simulink model "Autonomous_Driving_Car_Example1"  (R2022a)
settings: Solver=ode2  StartTime=0.0  StopTime=inf  FixedStep=1/600  RelTol=1e-3  EnableMultiTasking=on
model workspace (MAT data in the model file):
  camera_rate = Simulink.Parameter
  camera_rate.Value = Simulink.data.Expression
  camera_rate.Value.ExpressionString = "qc_get_step_size * ceil(1/60 / qc_get_step_size)"
  camera_rate.DataType = 'auto'
  camera_rate.Complexity = 'real'
  camera_rate.Dimensions = -1
  depth_rate = Simulink.Parameter
  depth_rate.Value = Simulink.data.Expression
  depth_rate.Value.ExpressionString = "qc_get_step_size * ceil(1/100 / qc_get_step_size)"
  depth_rate.DataType = 'auto'
  depth_rate.Complexity = 'real'
  depth_rate.Dimensions = -1
undefined symbols (not defined in the file): gcbh, height, HIL, JPEG, left, qc_get_step_size, top, Video3D, video_display_show, width
libraries: quarc_library x45, simulink x12
(part 1 of 2)
settings Model: SimulationMode=external  ExtModeTrigDuration=10000  Creator=User  LastModifiedBy=Admin
settings SolverCC: AlgebraicLoopSolver=TrustRegion  PositivePriorityOrder=on  AutoInsertRateTranBlk=on
settings DataIOCC: ReturnWorkspaceOutputs=off
settings DebuggingCC: ParameterPrecisionLossMsg=none  UnconnectedInputMsg=warning  UnconnectedOutputMsg=warning  UnconnectedLineMsg=warning  SFMachineParentedDataDiag=warning  ArithmeticOperatorsInVariantConditions=warning
settings HardwareCC: ProdBitPerLong=64  ProdLargestAtomicInteger=LongLong  ProdLargestAtomicFloat=Double  ProdLongLongMode=on  ProdHWDeviceType=ARM Compatible->ARM 64-bit (LP64)
settings SFSimCC: SimUseLocalCustomCode=off  CustomCodeUndefinedFunction=UseInterfaceOnly
settings RTWCC: Description=QUARC Linux Nvidia Target (QCar) Using Toolchain  SystemTargetFile=quarc_linux_nvidia.tlc  TemplateMakefile=quarc_default_tmf  RTWUseLocalCustomCode=off  Toolchain=QUARC linux_nvidia | gmake (64-bit Windows)  BuildConfiguration=Faster Runs
settings STFCustomTargetCC: TargetLangStandard=C99 (ISO)  ConcurrentExecutionCompliant=on  UseToolchainInfoCompliant=on  SystemTargetFile=quarc_linux_nvidia.tlc
settings GRTTargetCC: ParMdlRefBuildCompliant=off  CompOptLevelCompliant=off  CombineOutputUpdateFcns=off  MatFileLogging=off  CPPClassGenCompliant=off  GRTInterface=on  ExtMode=on  ExtModeMexFile=quarc_comm  ExtModeMexArgs='-w -d /tmp -uri %u','tcpip://192.168.2.11:17001'

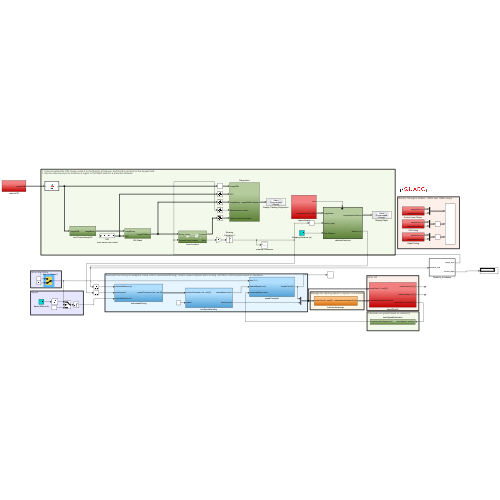
[thumbnail: Simulink's stored preview of the top-level diagram]
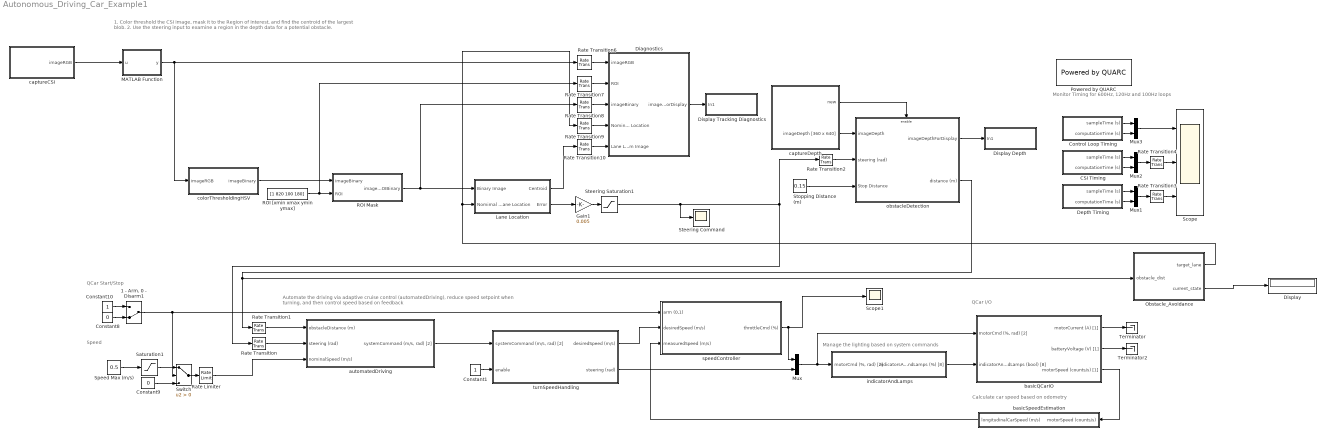
== system Autonomous_Driving_Car_Example1 ==
  note: Monitor Timing for 600Hz, 120Hz and 100Hz loops
  note: Manage the lighting based on system commands
  note: Calculate car speed based on odometry
  note: QCar I/O
  note: Automate the driving via adaptive cruise control (automatedDriving), reduce speed setpoint when turning, and then control speed based on feedback
  note: 1. Color threshold the CSI image, mask it to the Region of Interest, and find the centroid of the largest blob.
      | 2. Use the steering input to examine a region in the depth data for a potential obstacle.
  note: Speed
  note: QCar Start/Stop
  " CSI Timing" : Subsystem
  " Depth Timing" : Subsystem
  "1 - Arm, 0 - Disarm1" : ManualSwitch  CurrentSetting=0
  Constant1 : Constant
  Constant10 : Constant
  Constant8 : Constant  Value=0
  Constant9 : Constant  Value=0
  "Control Loop Timing " : Subsystem
  Diagnostics : Subsystem
  Display : Display
  Display Depth : Subsystem  LoadFcn=set_param(gcbh, 'UserData', gcb);  StartFcn=video_display_show([gcb, '/Video Display'], 'add', gcb);  mask(Video Compressed Display){algorithm=JPEG, quality=50, sample_time=-1, use_hardware=on}
      mask prompts: algorithm "Compression algorithm:"; quality "Compression quality (0-100):"; sample_time "Sample time (seconds):"; use_hardware "Use hardware acceleration for video display"
      mask help: Displays a video stream on the host, using compression to minimize bandwidth.
      mask init:
      | qc_set_display('Video\nCompressed\nDisplay');
      settings: UndoDeleteFcn=set_param(gcbh, 'UserData', gcb);  OpenFcn=video_display_show([gcb, '/Video Display'], 'show', gcb);  PreDeleteFcn=video_display_show([gcb, '/Video Display'], 'delete');
      settings: CopyFcn=|
      | set_param(gcbh, 'UserData', gcb);
      | set_param(gcbh, 'LinkStatus', 'none');
      settings: NameChangeFcn=|
      | video_display_show([get_param(gcbh, 'UserData'), '/Video Display'], 'rename', [gcb, '/Video Display']);
      | video_display_show([gcb, '/Video Display'], 'add', gcb);
      | set_param(gcbh, 'UserData', gcb);
      mask Help: web(qc_get_block_help_path(gcb));
      mask TypeOptions algorithm: Image Compress/algorithm
      mask TypeOptions quality: Image Compress/quality
      mask TypeOptions sample_time: Video Display/sample_time
      mask TypeOptions use_hardware: Video Display/use_hardware
      mask Display:
      | patch([0.98591 0.98591 0.62618 0.59072 0.56147   0.536   0.536  0.5441 0.56912 0.59207 0.60881 0.62276 0.63527 0.64364  0.6485  0.6485 0.64706 0.64499 0.63662 0.62411 0.61232 0.59837 0.58307 0.56147   0.536   0.536  0.5441  0.5747 0.60953 0.63662 0.67001  0.7034 0.72851 0.75425 0.77927 0.80294 0.82454 0.84119 0.85865 0.87395 0.88574 0.89339  0.8969 0.89969 0.89969 0.89267  0.8816 0.87044 0.85649  0.8384 0.81824 0.80294 0.78764 0.77513 0.76676 0.75776 0.76397 0.77513 0.79178 0.80987 0.82796 0.84326 0.86207 0.98528],[0.18689 0.05522 0.05522 0.05171 0.05171    0.05 0.18338 0.18338 0.19148 0.20435 0.22298 0.24863 0.28589 0.33125 0.38138 0.55139 0.59801 0.63761 0.68189 0.72149 0.74939 0.76694 0.77855 0.79367 0.79952 0.92768 0.92768 0.92768 0.92417 0.92066 0.91364  0.9032 0.89384 0.88106 0.86594 0.85073 0.82634 0.80537 0.77855 0.74363 0.70403 0.65858 0.61079 0.59099 0.41513 0.37202 0.31847 0.29048 0.25556 0.23342  0.2102 0.19382 0.18221 0.17285 0.16943 0.16124  0.1589 0.16241 0.16709 0.17168  0.1787 0.18221 0.18689 0.18689],[0.9,0.90,0.91])
      | patch([0.536 0.52601 0.46823 0.44528 0.41603 0.39101 0.35555 0.33116 0.31451 0.29291  0.2804 0.26717 0.25322 0.23999 0.22406 0.20732 0.19337 0.17528 0.15935 0.14396 0.13217 0.11759 0.10922 0.10085 0.09671 0.09392 0.09041 0.08906 0.08906 0.09464  0.0995 0.10778 0.11894 0.13145 0.14675 0.16349 0.17672 0.19409 0.20732 0.22406 0.23999 0.26159 0.27833 0.29849 0.31793 0.33602 0.35411 0.37085 0.39245 0.41603   0.536   0.536 0.53159 0.46409   0.446 0.42026 0.39587 0.37571 0.36113 0.34925 0.34088 0.33809 0.33809 0.34088 0.34583 0.35627 0.36392 0.38129 0.39587 0.41117 0.42719 0.44672  0.4676 0.48353 0.48353 0.52394   0.536],[0.05 0.04829 0.04712 0.04712 0.04829 0.05063 0.05405 0.05873 0.06107 0.06692 0.07043 0.07619 0.08087 0.08672 0.09482 0.10652 0.11696 0.13325  0.1508 0.17168 0.19499 0.22415 0.25439 0.28472 0.31379 0.35456 0.38489 0.41513 0.58055 0.63878 0.68774 0.72149 0.75641 0.78089 0.80537 0.82859 0.84029 0.85658 0.86594 0.87404  0.8834 0.89267 0.90086 0.90788 0.91247 0.91832 0.92066   0.923 0.92651 0.92768 0.92768 0.79952 0.79952 0.79952 0.79718 0.78899 0.77153 0.75056 0.72149 0.68072 0.62249  0.5549 0.41396 0.37085 0.33242 0.28121 0.25205 0.22181 0.20552 0.19499 0.18572 0.18221 0.17753 0.17636 0.17753  0.1787  0.1787],[0.9,0.90,0.91])
      | disp('Video\nCompressed\nDisplay');
  Display Tracking Diagnostics : Subsystem  LoadFcn=set_param(gcbh, 'UserData', gcb);  StartFcn=video_display_show([gcb, '/Video Display'], 'add', gcb);  mask(Video Compressed Display){algorithm=JPEG, quality=80, sample_time=-1, use_hardware=on}
      mask prompts: algorithm "Compression algorithm:"; quality "Compression quality (0-100):"; sample_time "Sample time (seconds):"; use_hardware "Use hardware acceleration for video display"
      mask help: Displays a video stream on the host, using compression to minimize bandwidth.
      mask init:
      | qc_set_display('Video\nCompressed\nDisplay');
      settings: UndoDeleteFcn=set_param(gcbh, 'UserData', gcb);  OpenFcn=video_display_show([gcb, '/Video Display'], 'show', gcb);  PreDeleteFcn=video_display_show([gcb, '/Video Display'], 'delete');
      settings: CopyFcn=|
      | set_param(gcbh, 'UserData', gcb);
      | set_param(gcbh, 'LinkStatus', 'none');
      settings: NameChangeFcn=|
      | video_display_show([get_param(gcbh, 'UserData'), '/Video Display'], 'rename', [gcb, '/Video Display']);
      | video_display_show([gcb, '/Video Display'], 'add', gcb);
      | set_param(gcbh, 'UserData', gcb);
      mask Help: web(qc_get_block_help_path(gcb));
      mask TypeOptions algorithm: Image Compress/algorithm
      mask TypeOptions quality: Image Compress/quality
      mask TypeOptions sample_time: Video Display/sample_time
      mask TypeOptions use_hardware: Video Display/use_hardware
      mask Display:
      | patch([0.98591 0.98591 0.62618 0.59072 0.56147   0.536   0.536  0.5441 0.56912 0.59207 0.60881 0.62276 0.63527 0.64364  0.6485  0.6485 0.64706 0.64499 0.63662 0.62411 0.61232 0.59837 0.58307 0.56147   0.536   0.536  0.5441  0.5747 0.60953 0.63662 0.67001  0.7034 0.72851 0.75425 0.77927 0.80294 0.82454 0.84119 0.85865 0.87395 0.88574 0.89339  0.8969 0.89969 0.89969 0.89267  0.8816 0.87044 0.85649  0.8384 0.81824 0.80294 0.78764 0.77513 0.76676 0.75776 0.76397 0.77513 0.79178 0.80987 0.82796 0.84326 0.86207 0.98528],[0.18689 0.05522 0.05522 0.05171 0.05171    0.05 0.18338 0.18338 0.19148 0.20435 0.22298 0.24863 0.28589 0.33125 0.38138 0.55139 0.59801 0.63761 0.68189 0.72149 0.74939 0.76694 0.77855 0.79367 0.79952 0.92768 0.92768 0.92768 0.92417 0.92066 0.91364  0.9032 0.89384 0.88106 0.86594 0.85073 0.82634 0.80537 0.77855 0.74363 0.70403 0.65858 0.61079 0.59099 0.41513 0.37202 0.31847 0.29048 0.25556 0.23342  0.2102 0.19382 0.18221 0.17285 0.16943 0.16124  0.1589 0.16241 0.16709 0.17168  0.1787 0.18221 0.18689 0.18689],[0.9,0.90,0.91])
      | patch([0.536 0.52601 0.46823 0.44528 0.41603 0.39101 0.35555 0.33116 0.31451 0.29291  0.2804 0.26717 0.25322 0.23999 0.22406 0.20732 0.19337 0.17528 0.15935 0.14396 0.13217 0.11759 0.10922 0.10085 0.09671 0.09392 0.09041 0.08906 0.08906 0.09464  0.0995 0.10778 0.11894 0.13145 0.14675 0.16349 0.17672 0.19409 0.20732 0.22406 0.23999 0.26159 0.27833 0.29849 0.31793 0.33602 0.35411 0.37085 0.39245 0.41603   0.536   0.536 0.53159 0.46409   0.446 0.42026 0.39587 0.37571 0.36113 0.34925 0.34088 0.33809 0.33809 0.34088 0.34583 0.35627 0.36392 0.38129 0.39587 0.41117 0.42719 0.44672  0.4676 0.48353 0.48353 0.52394   0.536],[0.05 0.04829 0.04712 0.04712 0.04829 0.05063 0.05405 0.05873 0.06107 0.06692 0.07043 0.07619 0.08087 0.08672 0.09482 0.10652 0.11696 0.13325  0.1508 0.17168 0.19499 0.22415 0.25439 0.28472 0.31379 0.35456 0.38489 0.41513 0.58055 0.63878 0.68774 0.72149 0.75641 0.78089 0.80537 0.82859 0.84029 0.85658 0.86594 0.87404  0.8834 0.89267 0.90086 0.90788 0.91247 0.91832 0.92066   0.923 0.92651 0.92768 0.92768 0.79952 0.79952 0.79952 0.79718 0.78899 0.77153 0.75056 0.72149 0.68072 0.62249  0.5549 0.41396 0.37085 0.33242 0.28121 0.25205 0.22181 0.20552 0.19499 0.18572 0.18221 0.17753 0.17636 0.17753  0.1787  0.1787],[0.9,0.90,0.91])
      | disp('Video\nCompressed\nDisplay');
  Gain1 : Gain  Gain=0.005
  Lane Location : Subsystem
  MATLAB Function : MATLAB Function  TreatAsAtomicUnit=on
  Mux{,1..3} (4 alike) : Mux  Inputs=2
  Obstacle_Avoidance : MATLAB Function  TreatAsAtomicUnit=on
  Powered by QUARC : quarc_library/Logos/Powered by QUARC
  ROI [xmin xmax ymin ymax] : Constant  Value=[1 820 100 180]
  ROI Mask : Subsystem
  Rate Limiter : RateLimiter  FallingSlewLimit=-Inf  SampleTimeMode=inherited
  Rate Transition{,1,3..4} (4 alike) : RateTransition
  Rate Transition{6..10} (5 alike) : RateTransition  OutPortSampleTime=0.1
  Rate Transition2 : RateTransition  Deterministic=off
  Saturation1 : Saturate  UpperLimit=1  LowerLimit=0
  Scope : Scope  NumInputPorts=3
  Scope1 : Scope
  Speed Max (m/s) : Constant  Value=0.5
  Steering Saturation1 : Saturate
  Steering Command : Scope
  Stopping Distance (m) : Constant  Value=0.15
  Switch : Switch  Criteria=u2 > Threshold  SaturateOnIntegerOverflow=off  InputSameDT=off
  Terminator : Terminator
  Terminator2 : Terminator
  automatedDriving : Subsystem
  basicQCarIO : Subsystem
  basicSpeedEstimation : Subsystem
  captureCSI : Subsystem
  captureDepth : Subsystem
  colorThresholdingHSV : Subsystem
  indicatorAndLamps : Subsystem
  obstacleDetection : Subsystem
  speedController : Subsystem
  turnSpeedHandling : Subsystem
  wires:
  Mux/1 -> basicQCarIO/1("motorCmd (%, rad) [2]"), indicatorAndLamps/1("motorCmd (%, rad) [2]")
  turnSpeedHandling/2(steering (rad)) -> Mux/2
  basicQCarIO/3(motorSpeed (counts/s) [1]) -> basicSpeedEstimation/1(motorSpeed (counts/s))
  basicSpeedEstimation/1(longitudinalCarSpeed (m/s)) -> speedController/3(measuredSpeed (m/s))
  basicQCarIO/1(motorCurrent (A) [1]) -> Terminator/1
  basicQCarIO/2(batteryVoltage (V) [1]) -> Terminator2/1
  Constant1/1 -> turnSpeedHandling/2(enable)
  indicatorAndLamps/1(indicatorsAndLamps (%) [8]) -> basicQCarIO/2(indicatorAndLamps (bool) [8])
  captureDepth/2(imageDepth [360 x 640]) -> obstacleDetection/1(imageDepth)
  automatedDriving/1("systemCommand (m/s, rad) [2]") -> turnSpeedHandling/1("systemCommand (m/s, rad) [2]")
  obstacleDetection/2(distance (m)) -> Rate Transition1/1, Obstacle_Avoidance/1(obstacle_dist)
  Rate Transition/1 -> automatedDriving/2(steering (rad))
  Rate Transition2/1 -> obstacleDetection/2(steering (rad))
  obstacleDetection/1(imageDepthForDisplay) -> Display Depth/1(In1)
  captureCSI/1(imageRGB) -> MATLAB Function/1(u)
  " Depth Timing"/2(computationTime (s)) -> Mux1/2
  " Depth Timing"/1(sampleTime (s)) -> Mux1/1
  " CSI Timing"/2(computationTime (s)) -> Mux2/2
  " CSI Timing"/1(sampleTime (s)) -> Mux2/1
  "Control Loop Timing "/2(computationTime (s)) -> Mux3/2
  "Control Loop Timing "/1(sampleTime (s)) -> Mux3/1
  Mux2/1 -> Rate Transition4/1
  Mux1/1 -> Rate Transition3/1
  Mux3/1 -> Scope/1
  Rate Transition3/1 -> Scope/3
  Rate Transition4/1 -> Scope/2
  captureDepth/1(new) -> obstacleDetection/Enable
  turnSpeedHandling/1(desiredSpeed (m/s)) -> speedController/2(desiredSpeed (m/s))
  Speed Max (m/s)/1 -> Saturation1/1
  Constant8/1 -> "1 - Arm, 0 - Disarm1"/2
  Saturation1/1 -> Switch/1
  Switch/1 -> Rate Limiter/1
  Constant10/1 -> "1 - Arm, 0 - Disarm1"/1
  "1 - Arm, 0 - Disarm1"/1 -> Switch/2, speedController/1(arm (0,1))
  Rate Limiter/1 -> automatedDriving/3(nominalSpeed (m/s))
  Constant9/1 -> Switch/3
  Steering Saturation1/1 -> Steering Command/1, Rate Transition/1, Rate Transition2/1
  Diagnostics/1(imageRGBForDisplay) -> Display Tracking Diagnostics/1(In1)
  ROI [xmin xmax ymin ymax]/1 -> Rate Transition7/1, ROI Mask/2(ROI)
  colorThresholdingHSV/1(imageBinary) -> ROI Mask/1(imageBinary)
  ROI Mask/1(imageROIBinary) -> Rate Transition8/1, Lane Location/1(Binary Image)
  Gain1/1 -> Steering Saturation1/1
  speedController/1(throttleCmd (%)) -> Scope1/1, Mux/1
  Rate Transition1/1 -> automatedDriving/1(obstacleDistance (m))
  Lane Location/1(Centroid) -> Rate Transition10/1
  Lane Location/2(Error) -> Gain1/1
  MATLAB Function/1(y) -> Rate Transition6/1, colorThresholdingHSV/1(imageRGB)
  Rate Transition6/1 -> Diagnostics/1(imageRGB)
  Rate Transition7/1 -> Diagnostics/2(ROI)
  Rate Transition8/1 -> Diagnostics/3(imageBinary)
  Rate Transition9/1 -> Diagnostics/4(Nominal Lane Location)
  Rate Transition10/1 -> Diagnostics/5(Lane Location from Image)
  Stopping Distance (m)/1 -> obstacleDetection/3(Stop Distance)
  Obstacle_Avoidance/1(target_lane) -> Rate Transition9/1, Lane Location/2(Nomimal Lane Location)
  Obstacle_Avoidance/2(current_state) -> Display/1

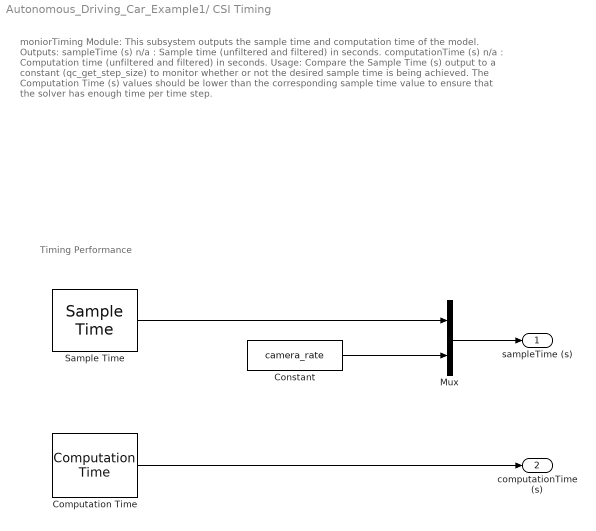
== system Autonomous_Driving_Car_Example1/ CSI Timing ==
  note: Timing Performance
  note: moniorTiming Module:
      |
      | This subsystem outputs the sample time and computation time of the model.
      |
      | Outputs:
      | sampleTime (s) n/a : Sample time (unfiltered and filtered) in seconds.
      | computationTime (s) n/a : Computation time (unfiltered and filtered) in seconds.
      |
      | Usage:
      | Compare the Sample Time (s) output to a constant (qc_get_step_size) to monitor whether or not the desired sample time is being achieved. The Computation Time (s) values should be lower than the corresponding sample time value to ensure that the solver has enough time per time step.
  Computation Time : quarc_library/Sources/Time/Computation Time  sample_time=camera_rate  use_model=on  use_cpu_time=off
  Constant : Constant  Value=camera_rate  SampleTime=camera_rate
  Mux : Mux  Inputs=2
  Sample Time : quarc_library/Sources/Time/Sample Time  Priority=-99  sample_time=camera_rate
  sampleTime (s) : Outport  VectorParamsAs1DForOutWhenUnconnected=off
  computationTime (s) : Outport  Port=2  VectorParamsAs1DForOutWhenUnconnected=off
  wires:
  Computation Time/1 -> computationTime (s)/1
  Mux/1 -> sampleTime (s)/1
  Sample Time/1 -> Mux/1
  Constant/1 -> Mux/2

== system Autonomous_Driving_Car_Example1/ Depth Timing ==
  note: moniorTiming Module:
      |
      | This subsystem outputs the sample time and computation time of the model.
      |
      | Outputs:
      | sampleTime (s) n/a : Sample time (unfiltered and filtered) in seconds.
      | computationTime (s) n/a : Computation time (unfiltered and filtered) in seconds.
      |
      | Usage:
      | Compare the Sample Time (s) output to a constant (qc_get_step_size) to monitor whether or not the desired sample time is being achieved. The Computation Time (s) values should be lower than the corresponding sample time value to ensure that the solver has enough time per time step.
  note: Timing Performance
  Computation Time : quarc_library/Sources/Time/Computation Time  sample_time=depth_rate  use_model=on  use_cpu_time=off
  Constant : Constant  Value=depth_rate  SampleTime=depth_rate
  Mux : Mux  Inputs=2
  Sample Time : quarc_library/Sources/Time/Sample Time  Priority=-99  sample_time=depth_rate
  sampleTime (s) : Outport  VectorParamsAs1DForOutWhenUnconnected=off
  computationTime (s) : Outport  Port=2  VectorParamsAs1DForOutWhenUnconnected=off
  wires:
  Constant/1 -> Mux/2
  Sample Time/1 -> Mux/1
  Mux/1 -> sampleTime (s)/1
  Computation Time/1 -> computationTime (s)/1

== system Autonomous_Driving_Car_Example1/Control Loop Timing  ==
  note: moniorTiming Module:
      |
      | This subsystem outputs the sample time and computation time of the model.
      |
      | Outputs:
      | sampleTime (s) n/a : Sample time (unfiltered and filtered) in seconds.
      | computationTime (s) n/a : Computation time (unfiltered and filtered) in seconds.
      |
      | Usage:
      | Compare the Sample Time (s) output to a constant (qc_get_step_size) to monitor whether or not the desired sample time is being achieved. The Computation Time (s) values should be lower than the corresponding sample time value to ensure that the solver has enough time per time step.
  note: Timing Performance
  Computation Time : quarc_library/Sources/Time/Computation Time  sample_time=qc_get_step_size  use_model=on  use_cpu_time=off
  Constant : Constant  Value=qc_get_step_size  SampleTime=-1
  Mux : Mux  Inputs=2
  Sample Time : quarc_library/Sources/Time/Sample Time  Priority=-99  sample_time=qc_get_step_size
  sampleTime (s) : Outport  VectorParamsAs1DForOutWhenUnconnected=off
  computationTime (s) : Outport  Port=2  VectorParamsAs1DForOutWhenUnconnected=off
  wires:
  Computation Time/1 -> computationTime (s)/1
  Constant/1 -> Mux/2
  Sample Time/1 -> Mux/1
  Mux/1 -> sampleTime (s)/1

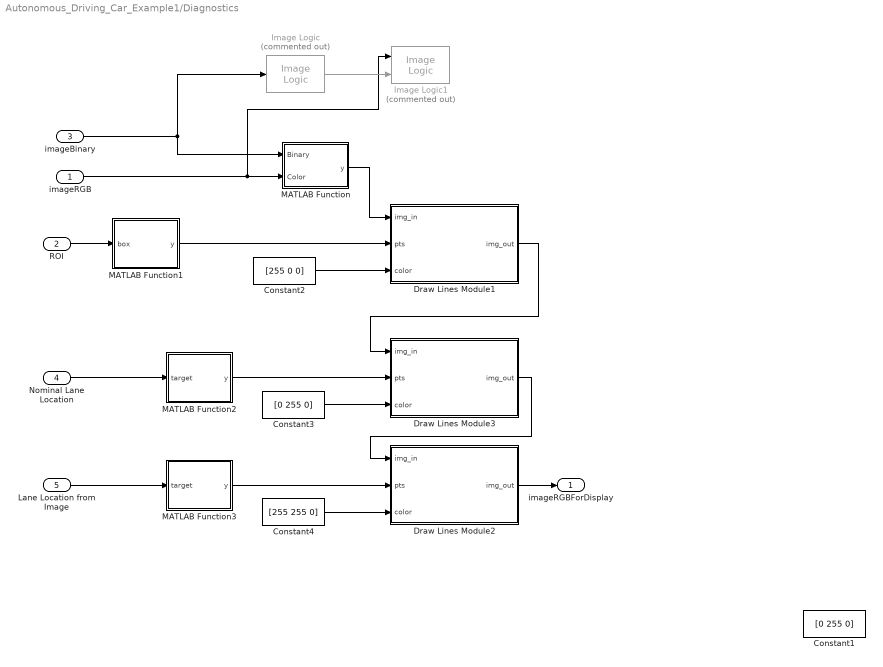
== system Autonomous_Driving_Car_Example1/Diagnostics ==
  imageRGB : Inport
  ROI : Inport  Port=2
  imageBinary : Inport  Port=3
  Nominal Lane Location : Inport  Port=4
  Lane Location from Image : Inport  Port=5
  Constant1 : Constant  Value=[0 255 0]
  Constant2 : Constant  Value=[255 0 0]
  Constant3 : Constant  Value=[0 255 0]
  Constant4 : Constant  Value=[255 255 0]
  Draw Lines Module1 : MATLAB Function  TreatAsAtomicUnit=on
  Draw Lines Module2 : MATLAB Function  TreatAsAtomicUnit=on
  Draw Lines Module3 : MATLAB Function  TreatAsAtomicUnit=on
  Image Logic : quarc_library/Image Processing/Generic/Image Logic  Commented=on  algorithm=NOT  source=Internal dialog parameter  row=0  column=0
      settings: AttributesFormatString=(%<algorithm>)  SourceProductName=QUARC Targets
  Image Logic1 : quarc_library/Image Processing/Generic/Image Logic  Commented=on  algorithm=AND  source=Internal dialog parameter  row=0  column=0
      settings: AttributesFormatString=(%<algorithm>)  SourceProductName=QUARC Targets
  MATLAB Function : MATLAB Function  TreatAsAtomicUnit=on
  MATLAB Function1 : MATLAB Function  TreatAsAtomicUnit=on
  MATLAB Function2 : MATLAB Function  TreatAsAtomicUnit=on
  MATLAB Function3 : MATLAB Function  TreatAsAtomicUnit=on
  imageRGBForDisplay : Outport  VectorParamsAs1DForOutWhenUnconnected=off
  wires:
  Constant2/1 -> Draw Lines Module1/3(color)
  imageRGB/1 -> Image Logic1/1, MATLAB Function/2(Color)
  MATLAB Function1/1(y) -> Draw Lines Module1/2(pts)
  ROI/1 -> MATLAB Function1/1(box)
  Draw Lines Module3/1(img_out) -> Draw Lines Module2/1(img_in)
  Draw Lines Module1/1(img_out) -> Draw Lines Module3/1(img_in)
  Constant3/1 -> Draw Lines Module3/3(color)
  MATLAB Function2/1(y) -> Draw Lines Module3/2(pts)
  Nominal Lane Location/1 -> MATLAB Function2/1(target)
  imageBinary/1 -> MATLAB Function/1(Binary), Image Logic/1
  MATLAB Function/1(y) -> Draw Lines Module1/1(img_in)
  Lane Location from Image/1 -> MATLAB Function3/1(target)
  MATLAB Function3/1(y) -> Draw Lines Module2/2(pts)
  Constant4/1 -> Draw Lines Module2/3(color)
  Image Logic/1 -> Image Logic1/2
  Draw Lines Module2/1(img_out) -> imageRGBForDisplay/1

== system Autonomous_Driving_Car_Example1/Display Depth ==
  In1 : Inport
  Channel : quarc_library/Signal Routing/Channel  channel=0  buffer_size=1
  Image Compress : quarc_library/Image Processing/Generic/Image Compress  algorithm=JPEG  source=Internal dialog parameter  quality=quality  output_dim=-1
  Video Display : quarc_library/Multimedia/Video Display  Tag=Autonomous_Driving_Car_Example1/Display Depth/Video Display  sample_time=sample_time  use_hardware=on
  wires:
  Channel/1 -> Video Display/1
  In1/1 -> Image Compress/1
  Image Compress/1 -> Channel/1

== system Autonomous_Driving_Car_Example1/Display Tracking Diagnostics ==
  In1 : Inport
  Channel : quarc_library/Signal Routing/Channel  channel=1  buffer_size=1
  Image Compress : quarc_library/Image Processing/Generic/Image Compress  algorithm=JPEG  source=Internal dialog parameter  quality=quality  output_dim=-1
  Video Display : quarc_library/Multimedia/Video Display  Tag=Autonomous_Driving_Car_Example1/Display Tracking Diagnostics/Video Display  sample_time=sample_time  use_hardware=on
  wires:
  Channel/1 -> Video Display/1
  In1/1 -> Image Compress/1
  Image Compress/1 -> Channel/1

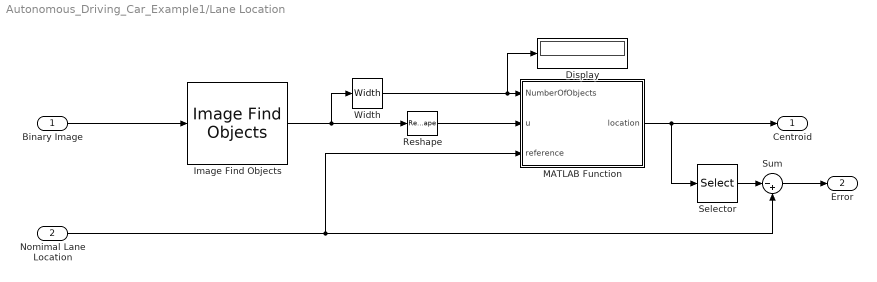
== system Autonomous_Driving_Car_Example1/Lane Location ==
  Binary Image : Inport
  Nomimal Lane Location : Inport  Port=2
  Display : Display
  Image Find Objects : quarc_library/Image Processing/Generic/Image Find Objects  num_objects=1  connectivity=4 directions (N, E, S, W)  sort_order=Sort by number of pixels  min_pixels=50  max_pixels=intmax('uint32')  largest=on  exclude_at_edges=off  variable_size=on  use_complex=off
      settings: SourceProductName=QUARC Targets
  MATLAB Function : MATLAB Function  TreatAsAtomicUnit=on
  Reshape : Reshape
  Selector : Selector  InputPortWidth=2  IndexOptions=Index vector (dialog)  Indices=[2]  OutputSizes=1
  Sum : Sum  Inputs=|-+
  Width : Width
  Centroid : Outport  VectorParamsAs1DForOutWhenUnconnected=off
  Error : Outport  Port=2  VectorParamsAs1DForOutWhenUnconnected=off
  wires:
  Binary Image/1 -> Image Find Objects/1
  Image Find Objects/3 -> Width/1, Reshape/1
  Nomimal Lane Location/1 -> Sum/2, MATLAB Function/3(reference)
  MATLAB Function/1(location) -> Selector/1, Centroid/1
  Width/1 -> Display/1, MATLAB Function/1(NumberOfObjects)
  Reshape/1 -> MATLAB Function/2(u)
  Selector/1 -> Sum/1
  Sum/1 -> Error/1

== system Autonomous_Driving_Car_Example1/ROI Mask ==
  note: HSV-Color Thresholding Module:
      |
      | This subsystem thresholds a given RGB image based on the desired colour and hue
      |
      | Inputs:
      | imageRGB (uint8) {0,255} : Input RGB Image to be thresholded
      | desiredHue (int) {-1}U{0,360} : Desired Hue to threshold around (provided in the 0-360 degree range, see the color wheel for hue selection)
      | Set the desired hue to -1 if you are interested in thresholding for white
      | [Sat_min, Val_min] (uint8) {0,255} : Minimum Saturation and Value thresholds
      | [Sat_max, Val_max] (uint8) {0,255} : Maximum Saturation and Value thresholds
      |
      | Outputs:
      | imageBinary (uint8) {0,255} : Binary Image (0 or 255 and no other value) representing the thresholding output
      |
      | Usage:
      | This module can be used when you are interested in thresholding for a certain hue regardless of the luminance. Compared to RGB thresholding which does not work well when the lighting conditions vary, HSV thresholding will correctly threshold for a hue (color) and allow you to specify a broad range of illuminance via the saturation and value thresholds. To broaden the range of hues accepted in the thresholding block, increase the Hue Threshold parameter.
  imageBinary : Inport
  ROI : Inport  Port=2
  Image Logic2 : quarc_library/Image Processing/Generic/Image Logic  algorithm=AND  source=Internal dialog parameter  row=0  column=0
      settings: AttributesFormatString=(%<algorithm>)  SourceProductName=QUARC Targets
  Mask : MATLAB Function  TreatAsAtomicUnit=on
  imageROIBinary : Outport  VectorParamsAs1DForOutWhenUnconnected=off
  wires:
  imageBinary/1 -> Image Logic2/1
  Image Logic2/1 -> imageROIBinary/1
  ROI/1 -> Mask/1(box)
  Mask/1(y) -> Image Logic2/2

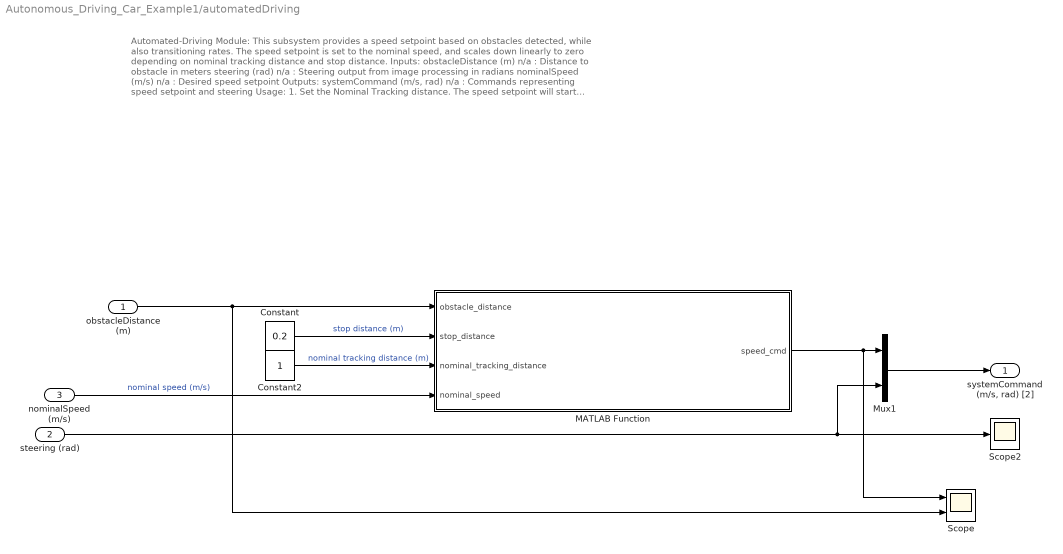
== system Autonomous_Driving_Car_Example1/automatedDriving ==
  note: Automated-Driving Module:
      |
      | This subsystem provides a speed setpoint based on obstacles detected, while also transitioning rates. The speed setpoint is set to the nominal speed, and scales down linearly to zero depending on nominal tracking distance and stop distance.
      |
      | Inputs:
      | obstacleDistance (m) n/a : Distance to obstacle in meters
      | steering (rad) n/a : Steering output from image processing in radians
      | nominalSpeed (m/s) n/a : Desired speed setpoint
      |
      | Outputs:
      | systemCommand (m/s, rad) n/a : Commands representing speed setpoint and steering
      |
      | Usage:
      | 1. Set the Nominal Tracking distance. The speed setpoint will start decreasing if the obstacle distance is less than this threshold.
      | 2. Set the Stop Distance. The speed setpoint will scale down to 0 when the the obstacle distance reaches this threshold.
  obstacleDistance (m) : Inport
  steering (rad) : Inport  Port=2
  nominalSpeed (m/s) : Inport  Port=3
  Constant : Constant  Value=0.2
  Constant2 : Constant
  MATLAB Function : MATLAB Function  TreatAsAtomicUnit=on
  Mux1 : Mux  Inputs=2
  Scope : Scope  NumInputPorts=2
  Scope2 : Scope
  "systemCommand (m/s, rad) [2]" : Outport  VectorParamsAs1DForOutWhenUnconnected=off
  wires:
  nominalSpeed (m/s)/1 -> MATLAB Function/4(nominal_speed)  "nominal speed (m/s)"
  Constant2/1 -> MATLAB Function/3(nominal_tracking_distance)  "nominal tracking distance (m)"
  Constant/1 -> MATLAB Function/2(stop_distance)  "stop distance (m)"
  MATLAB Function/1(speed_cmd) -> Scope/1, Mux1/1
  steering (rad)/1 -> Mux1/2, Scope2/1
  Mux1/1 -> "systemCommand (m/s, rad) [2]"/1
  obstacleDistance (m)/1 -> Scope/2, MATLAB Function/1(obstacle_distance)

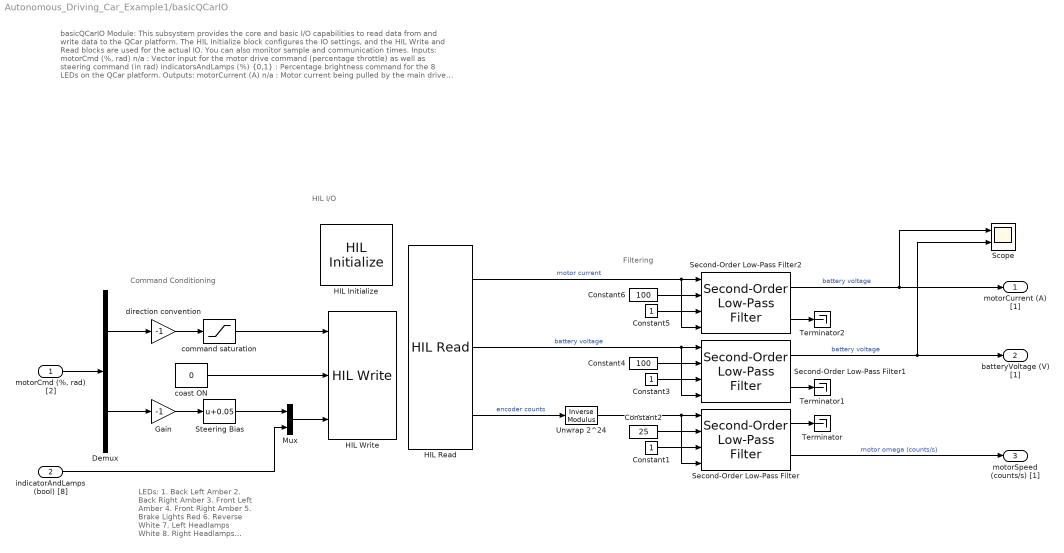
== system Autonomous_Driving_Car_Example1/basicQCarIO ==
  note: Filtering
  note: basicQCarIO Module:
      |
      | This subsystem provides the core and basic I/O capabilities to read data from and write data to the QCar platform. The HIL Initialize block configures the IO settings, and the HIL Write and Read blocks are used for the actual IO. You can also monitor sample and communication times.
      |
      | Inputs:
      | motorCmd (%, rad) n/a : Vector input for the motor drive command (percentage throttle) as well as steering command (in rad)
      | indicatorsAndLamps (%) {0,1} : Percentage brightness command for the 8 LEDs on the QCar platform.
      |
      | Outputs:
      | motorCurrent (A) n/a : Motor current being pulled by the main drive motor
      | batteryVoltage (V) {0, 12.6} : Current battery voltage reading
      | motorSpeed (counts/s) n/a : Drive motor speed measured using an encoder (do not confuse with wheel speed as this measurement is at the drive shaft)
  note: Command Conditioning
  note: HIL I/O
  note: LEDs:
      | 1. Back Left Amber
      | 2. Back Right Amber
      | 3. Front Left Amber
      | 4. Front Right Amber
      | 5. Brake Lights Red
      | 6. Reverse White
      | 7. Left Headlamps White
      | 8. Right Headlamps White
  "motorCmd (%, rad) [2]" : Inport
  indicatorAndLamps (bool) [8] : Inport  Port=2
  Constant1 : Constant
  Constant2 : Constant  Value=25
  Constant3 : Constant
  Constant4 : Constant  Value=100
  Constant5 : Constant
  Constant6 : Constant  Value=100
  Demux : Demux  Outputs=2
  Gain : Gain  Gain=-1
  HIL Initialize : quarc_library/Data Acquisition/Generic/Configuration/HIL Initialize  object_name=HIL-1  board_type=qcar  board_number=0  board_options=gyro_fs=250;gyro_rate=64;accel_fs=2;accel_rate=62.5;mag_rate=20;mag_xy=47;mag_z=83;enc1_dir=0;enc2_dir=0;enc3_dir=0;enc4_dir=0;pwm1_dshot=0;pwm2_dshot=0;pwm3_dshot=0;pwm4_dshot=0;pwm5_dshot=0;pwm6_dshot=0;pwm7_dshot=0;steer_bias=0.05;motor_limit=0.3;  exclusive=off  active=on  hardware_clocks=[]  clock_modes=[]  initial_clock_frequencies=[]  set_clock_params_at_start=off  set_clock_params_at_switch_in=off  set_clock_frequencies_at_start=off  set_clock_frequencies_at_switch_in=off  analog_input_channels=[0:6]  analog_input_configurations=[]  analog_input_maximums=[3.3]  analog_input_minimums=[0]  set_analog_input_params_at_start=off  set_analog_input_params_at_switch_in=off  analog_output_channels=[]  analog_output_maximums=[]  analog_output_minimums=[]  initial_analog_outputs=[]  final_analog_outputs=[]  watchdog_analog_outputs=[]  set_analog_output_params_at_start=off  set_analog_output_params_at_switch_in=off  set_analog_outputs_at_start=off  set_analog_outputs_at_switch_in=off  set_analog_outputs_at_terminate=off  set_analog_outputs_at_switch_out=off  set_analog_outputs_on_watchdog=off  digital_input_channels=[24:43]  digital_output_channels=[40]  digital_output_configuration=[]  initial_digital_outputs=[0]  final_digital_outputs=[1]  watchdog_digital_outputs=[]  set_digital_output_params_at_start=off  set_digital_output_params_at_switch_in=off  set_digital_outputs_at_start=on  set_digital_outputs_at_switch_in=off  set_digital_outputs_at_terminate=on  set_digital_outputs_at_switch_out=off  set_digital_outputs_on_watchdog=off  encoder_channels=[0:4]  quadrature=[4 4]  encoder_filter_frequency=100e6/1  initial_encoder_counts=[0]  set_encoder_params_at_start=on  set_encoder_params_at_switch_in=off  set_encoder_counts_at_start=on  set_encoder_counts_at_switch_in=off  pwm_channels=[0:7]  pwm_modes=[0 0]  pwm_frequency=150e6/4096  pwm_configuration=[0]  pwm_alignment=[0]  pwm_polarity=[1]  pwm_leading_deadband=[]  pwm_trailing_deadband=[]  initial_pwm_outputs=[0]  final_pwm_outputs=[0]  watchdog_pwm_outputs=[0]  set_pwm_params_at_start=on  set_pwm_params_at_switch_in=off  set_pwm_outputs_at_start=on  set_pwm_outputs_at_switch_in=off  set_pwm_outputs_at_terminate=on  set_pwm_outputs_at_switch_out=off  set_pwm_outputs_on_watchdog=off  other_output_channels=[1000, 11000:11011]  initial_other_outputs=[0]  final_other_outputs=[0]  watchdog_other_outputs=[]  set_other_outputs_at_start=on  set_other_outputs_at_switch_in=off  set_other_outputs_at_terminate=on  set_other_outputs_at_switch_out=off  set_other_outputs_on_watchdog=off
  HIL Read : quarc_library/Data Acquisition/Generic/Immediate I//O/HIL Read  object_name=HIL-1  analog_channels=[5:6]  encoder_channels=[0]  digital_channels=[]  other_channels=[]  sample_time=qc_get_step_size  active=on  vector_output=off  data_type_mode=Inherit via back propagation  encoder_data_type=double  digital_data_type=boolean
  HIL Write : quarc_library/Data Acquisition/Generic/Immediate I//O/HIL Write  object_name=HIL-1  analog_channels=[]  pwm_channels=[0]  digital_channels=[40]  other_channels=[1000 11008:11011 11000:11003]  sample_time=qc_get_step_size  active=off  vector_input=on
  Mux : Mux  Inputs=2
  Scope : Scope  NumInputPorts=2
  Second-Order Low-Pass Filter : quarc_library/Continuous/Second-Order Low-Pass Filter  params_source=External (input ports)  input_width=1  input_zeta=1  input_init=0
  Second-Order Low-Pass Filter1 : quarc_library/Continuous/Second-Order Low-Pass Filter  params_source=External (input ports)  input_width=1  input_zeta=1  input_init=0
  Second-Order Low-Pass Filter2 : quarc_library/Continuous/Second-Order Low-Pass Filter  params_source=External (input ports)  input_width=1  input_zeta=1  input_init=0
  Steering Bias : Bias  Bias=0.05  SaturateOnIntegerOverflow=off
  Terminator : Terminator
  Terminator1 : Terminator
  Terminator2 : Terminator
  Unwrap 2^24 : quarc_library/Discontinuities/Inverse Modulus  modulus=16777215  output_derivative=off  output_revolutions=off  max_x=Inf  min_x=-Inf
  coast ON : Constant  Value=0
  command saturation : Saturate  UpperLimit=0.25  LowerLimit=-0.25
  direction convention : Gain  Gain=-1
  motorCurrent (A) [1] : Outport  VectorParamsAs1DForOutWhenUnconnected=off
  batteryVoltage (V) [1] : Outport  Port=2  VectorParamsAs1DForOutWhenUnconnected=off
  motorSpeed (counts/s) [1] : Outport  Port=3  VectorParamsAs1DForOutWhenUnconnected=off
  wires:
  Second-Order Low-Pass Filter2/1 -> Scope/1, motorCurrent (A) [1]/1  "battery voltage"
  Constant2/1 -> Second-Order Low-Pass Filter/2
  Unwrap 2^24/1 -> Second-Order Low-Pass Filter/1, Second-Order Low-Pass Filter/4
  Demux/2 -> Gain/1
  direction convention/1 -> command saturation/1
  "motorCmd (%, rad) [2]"/1 -> Demux/1
  command saturation/1 -> HIL Write/1
  Second-Order Low-Pass Filter/1 -> Terminator/1
  Constant3/1 -> Second-Order Low-Pass Filter1/3
  indicatorAndLamps (bool) [8]/1 -> Mux/2
  Steering Bias/1 -> Mux/1
  Second-Order Low-Pass Filter1/1 -> Scope/2, batteryVoltage (V) [1]/1  "battery voltage"
  Constant5/1 -> Second-Order Low-Pass Filter2/3
  Second-Order Low-Pass Filter1/2 -> Terminator1/1
  HIL Read/2 -> Second-Order Low-Pass Filter1/1, Second-Order Low-Pass Filter1/4  "battery voltage"
  Mux/1 -> HIL Write/3
  Constant6/1 -> Second-Order Low-Pass Filter2/2
  Second-Order Low-Pass Filter/2 -> motorSpeed (counts/s) [1]/1  "motor omega (counts/s)"
  Second-Order Low-Pass Filter2/2 -> Terminator2/1
  Constant4/1 -> Second-Order Low-Pass Filter1/2
  Constant1/1 -> Second-Order Low-Pass Filter/3
  Demux/1 -> direction convention/1
  HIL Read/3 -> Unwrap 2^24/1  "encoder counts"
  HIL Read/1 -> Second-Order Low-Pass Filter2/1, Second-Order Low-Pass Filter2/4  "motor current"
  Gain/1 -> Steering Bias/1
  coast ON/1 -> HIL Write/2

== system Autonomous_Driving_Car_Example1/basicSpeedEstimation ==
  note: speedEstimation Module:
      |
      | This subsystem converts the motor speed measurements in counts/s to a useful longitudinal car speed in m/s.
      |
      | Inputs:
      | motorSpeed (counts/s) n/a : Drive motor speed measured using an encoder
      |
      | Outputs:
      | longitudinalCarSpeed (m/s) n/a : The platform's longitudinal speed (along the front-rear axis direction)
  note: (Diff. pinion*pinion)/(Spur*Diff. spur)
  note: v = 2*pi*r * omega (if omega is in rot/s)
      | v = r * omega (if omega is in rad/s)
      | r = 0.0342 m
  note: Estimate car speed from motor encoder counts rate
  motorSpeed (counts/s) : Inport
  counts to rotations : Gain  Gain=1/720/4
  gear ratios : Gain  Gain=(13*19)/(70*37)
  rot/s to rad/s : Gain  Gain=2*pi
  wheel radius : Gain  Gain=0.0342
  longitudinalCarSpeed (m/s) : Outport  VectorParamsAs1DForOutWhenUnconnected=off
  wires:
  gear ratios/1 -> rot/s to rad/s/1  "shaft speed (rots/s)"
  wheel radius/1 -> longitudinalCarSpeed (m/s)/1  "wheel speed (m/s)"
  counts to rotations/1 -> gear ratios/1  "motor speed (rot/s)"
  rot/s to rad/s/1 -> wheel radius/1  "wheel speed (rad/s)"
  motorSpeed (counts/s)/1 -> counts to rotations/1

== system Autonomous_Driving_Car_Example1/captureCSI ==
  note: Capture CSI RGB Information at 120 fps, 820 x 410
  note: captureCSI Module:
      |
      | This subsystem outputs the RGB Image captured from the associated CSI device
      |
      | Outputs:
      | RGB (uint8) : RGB Image [height, width, 3]
      | new (bool) : Boolean flag that is high (1) when the data is new
      |
      | Usage:
      | Double-click the Video Capture block and set the 'Device Identifier' parameter to the desired value.
      | Also set the desired resolution and frame rate.
      |
      | Sample Rate:
      | The sample rate for this model is defined as the model workspace variable camera_rate found under the Model Explorer/Model Workspace . For this subsystem the image acquisition is done at a rate of 120 Hz.
  Scope : Scope
  Video Capture : quarc_library/Multimedia/Video Capture  source=device  device=3  filename=sample_movie.mov  value=[0 0; 0 0]  resolution=820 x 410  width=820  height=410  output_format=MATLAB RGB (HxWx3)  data_type=uint8  sample_time=camera_rate  brightness_override=off  brightness=50.0  contrast_override=off  contrast=50.0  hue_override=off  hue=50.0  saturation_override=off  saturation=50.0  sharpness_override=off  sharpness=50.0  gamma_override=off  gamma=50.0  coloreffect_override=off  coloreffect=None  whitebalance_override=off  whitebalance=50.0  backlightcompensation_override=off  backlightcompensation=0.0  gain_override=off  gain=50.0  pan_override=off  pan=50.0  tilt_override=off  tilt=50.0  roll_override=off  roll=50.0  zoom_override=off  zoom=0.0  exposure_override=off  exposure=50.0  iris_override=off  iris=50.0  focus_override=off  focus=0.0
      settings: SourceProductName=QUARC Targets
  imageRGB : Outport  VectorParamsAs1DForOutWhenUnconnected=off
  wires:
  Video Capture/1 -> imageRGB/1
  Video Capture/2 -> Scope/1

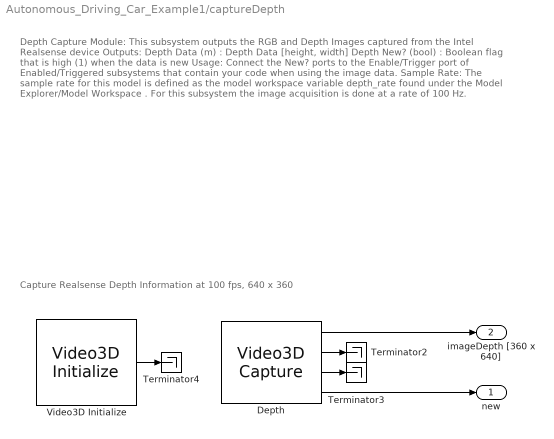
== system Autonomous_Driving_Car_Example1/captureDepth ==
  note: Depth Capture Module:
      |
      | This subsystem outputs the RGB and Depth Images captured from the Intel Realsense device
      |
      | Outputs:
      | Depth Data (m) : Depth Data [height, width]
      | Depth New? (bool) : Boolean flag that is high (1) when the data is new
      |
      | Usage:
      | Connect the New? ports to the Enable/Trigger port of Enabled/Triggered subsystems that contain your code when using the image data.
      |
      | Sample Rate:
      | The sample rate for this model is defined as the model workspace variable depth_rate found under the Model Explorer/Model Workspace . For this subsystem the image acquisition is done at a rate of 100 Hz.
  note: Capture Realsense Depth Information at 100 fps, 640 x 360
  Depth : quarc_library/Multimedia/Video3D Capture  object_name=Video3D-1  stream_type=Depth  stream_index=0  resolution=640 x 360  width=640  height=360  output_format=Distance in meters (HxW)  data_type=single  sample_time=depth_rate  camera_intrinsics=off  depth_scale=off  brightness_override=off  brightness=50.0  contrast_override=off  contrast=50.0  hue_override=off  hue=50.0  saturation_override=off  saturation=50.0  sharpness_override=off  sharpness=50.0  gamma_override=off  gamma=50.0  gain_override=off  gain=50.0  backlightcompensation_override=off  backlightcompensation=50.0  whitebalance_override=Automatic white balance  whitebalance=50.0  exposure_override=Automatic exposure  exposure=30.0  emitter=Enable laser emitter  preset=Do not set camera presets
  Terminator2 : Terminator
  Terminator3 : Terminator
  Terminator4 : Terminator
  Video3D Initialize : quarc_library/Multimedia/Video3D Initialize  object_name=Video3D-1  source=Device  identifier=0  file=sample.bag  sample_time=depth_rate  active=on
  new : Outport  VectorParamsAs1DForOutWhenUnconnected=off
  imageDepth [360 x 640] : Outport  Port=2  VectorParamsAs1DForOutWhenUnconnected=off
  wires:
  Depth/4 -> new/1
  Depth/1 -> imageDepth [360 x 640]/1
  Video3D Initialize/1 -> Terminator4/1
  Depth/3 -> Terminator3/1
  Depth/2 -> Terminator2/1
